simulink model "dynamic_of_reaction_wheel"  (R2025a)
settings: Solver=VariableStepAuto  StartTime=0.0  StopTime=10  RelTol=1e-3
InitFcn:
  | run(fullfile(fileparts(get_param(bdroot,'FileName')),'Params.m'));
values from neighbouring files (symbols this model uses):
  bc = 0    [Params.m]
  body_accel_gain = 1/IcO_bar    [Params.m]
  bw = 1.06e-5    (= 1.06e-05)    [Params.m]
  cd = 1.70e-8    (= 1.7e-08)    [Params.m]
  com_angle_offset = 0    [Params.m]
  gravity_gain = mtot*g*d    [Params.m]
  tau_c = 2.46e-3    (= 0.00246)    [Params.m]
  tau_input = 0    [Params.m]
  thetab0 = deg2rad(45)    [Params.m]
  thetabdot0 = 0    [Params.m]
  thetaw0 = 0    [Params.m]
  thetawdot0 = 0    [Params.m]
  w_eps = 0.5    [Params.m]
  wheel_accel_gain = 1/Iwg    (= 8000)    [Params.m]
settings Model: NumberOfSteps=5  Creator=Tran Anh Duy  LastModifiedBy=Tran Anh Duy

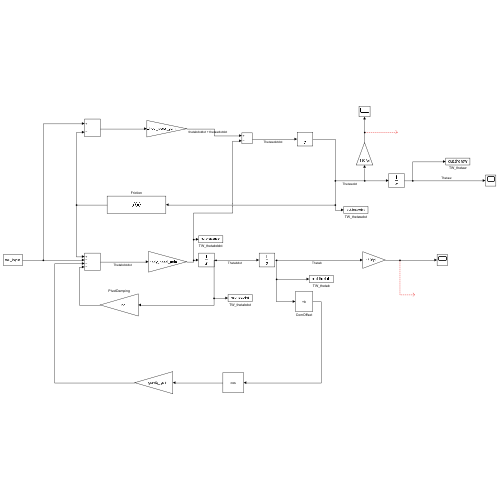
[thumbnail: Simulink's stored preview of the top-level diagram]
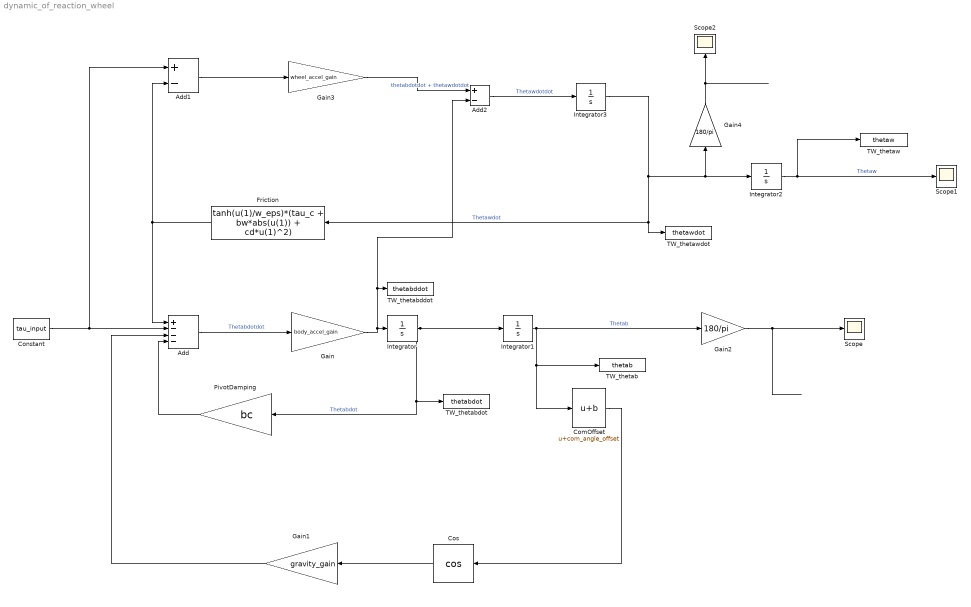
== system dynamic_of_reaction_wheel ==
  Add : Sum  Inputs=+---
  Add1 : Sum  Inputs=+-
  Add2 : Sum  Inputs=+-
  ComOffset : Bias  Bias=com_angle_offset  SaturateOnIntegerOverflow=off
  Constant : Constant  Value=tau_input
  Cos : Trigonometry  Operator=cos
  Friction : Fcn  Expr=tanh(u(1)/w_eps)*(tau_c + bw*abs(u(1)) + cd*u(1)^2)
  Gain : Gain  Gain=body_accel_gain
  Gain1 : Gain  Gain=gravity_gain
  Gain2 : Gain  Gain=180/pi
  Gain3 : Gain  Gain=wheel_accel_gain
  Gain4 : Gain  Gain=180/pi
  Integrator : Integrator  InitialCondition=thetabdot0
  Integrator1 : Integrator  InitialCondition=thetab0
  Integrator2 : Integrator  InitialCondition=thetaw0
  Integrator3 : Integrator  InitialCondition=thetawdot0
  PivotDamping : Gain  Gain=bc
  Scope : Scope
      settings: ActiveDisplayYMinimum=-306.16974277571381  ActiveDisplayYMaximum=134.01886030841263
  Scope1 : Scope
      settings: ActiveDisplayYMinimum=-3.0458122917304919  ActiveDisplayYMaximum=2.4537539479135297
  Scope2 : Scope
      settings: ActiveDisplayYMinimum=-815.06997909597271  ActiveDisplayYMaximum=740.6128624716132  DataLoggingVariableName=ScopeData2
  TW_thetab : ToWorkspace  VariableName=thetab  SaveFormat=Timeseries  SampleTime=-1
  TW_thetabddot : ToWorkspace  VariableName=thetabddot  SaveFormat=Timeseries  SampleTime=-1
  TW_thetabdot : ToWorkspace  VariableName=thetabdot  SaveFormat=Timeseries  SampleTime=-1
  TW_thetaw : ToWorkspace  VariableName=thetaw  SaveFormat=Timeseries  SampleTime=-1
  TW_thetawdot : ToWorkspace  VariableName=thetawdot  SaveFormat=Timeseries  SampleTime=-1
  wires:
  Add/1 -> Gain/1  "Thetabdotdot"
  Gain/1 -> Add2/2, TW_thetabddot/1, Integrator/1
  Integrator/1 -> PivotDamping/1, TW_thetabdot/1, Integrator1/1  "Thetabdot"
  Integrator1/1 -> ComOffset/1, TW_thetab/1, Gain2/1  "Thetab"
  Gain1/1 -> Add/3
  Constant/1 -> Add1/1, Add/2
  Integrator3/1 -> TW_thetawdot/1, Friction/1, Integrator2/1, Gain4/1  "Thetawdot"
  Integrator2/1 -> Scope1/1, TW_thetaw/1  "Thetaw"
  Add1/1 -> Gain3/1
  Cos/1 -> Gain1/1
  Gain2/1 -> Scope/1
  Gain4/1 -> Scope2/1
  Gain3/1 -> Add2/1  "thetabdotdot + thetawdotdot"
  Add2/1 -> Integrator3/1  "Thetawdotdot"
  Friction/1 -> Add1/2, Add/1
  ComOffset/1 -> Cos/1
  PivotDamping/1 -> Add/4
